simulink model "heli_p4_kalman_kf_r2020b"  (R2020b)
settings: Solver=ode1  StartTime=0.0  StopTime=45  FixedStep=0.002  RelTol=1e-3  EnableMultiTasking=on
PostLoadFcn:
  | qc_set_target_type(getConfigSet(bdroot, 'QUARC Default Target Configuration'));
values from neighbouring files (symbols this model uses):
  Ad = sys_kf.A    [p4_kalman.m]
  Bd = sys_kf.B    [p4_kalman.m]
  Cd = sys_kf.C    [p4_kalman.m]
  e_offset = heli_e_offset()    [heli_params.m]
  F = zeros(2)    [p4_controller.m]    (also in p4_kalman.m = zeros(size(F)))
  Joystick_gain_x = 1    [init_heli_3_10.m]
  Joystick_gain_y = -1    [init_heli_3_10.m]
  K = lqr(A_lqri, B_lqri, Q, R)    [p4_controller.m]    (also in p4_kalman.m = zeros(size(K)); p4_report_figs.m = floor((numel(x) - N)/step) + 1; p4_report_figs_backup_20261114.m = floor((numel(x) - N)/step) + 1; p4_report_figs_backup_before_qd_limits.m = floor((numel(x) - N)/step) + 1)
  P0 = eye(6)    [p4_kalman.m]
  Qd = Qd_vl    [p4_kalman.m]
  Rd = [0.00131511792463 0.00165099561417 0.00239206219708 -0.000707556992436 -6.43652106551e-05 0.00165099561417 0.0114715333934 0.0157536439693 -0.00145108778115 -0.000320746387433 0.00239206219708 0.0157536439693 ... (25 elements, 5x5)]    [Rd_flying.mat]    (also in p4_kalman.m = diag([1e-3 1e-3 1e-3 1e-3 1e-3]); p4_noise.m = R_hover)
  Vs0 = 7.3    [heli_params.m]    (also in p4_kalman.m = 0)
  x0 = zeros(6,1)    [p4_kalman.m]
undefined symbols (not defined in the file or in its folder): HIL, qc_get_step_size
libraries: quarc_library x9
settings Model: SimulationMode=external  ExtModeTrigDuration=60000  Creator=Rchan  LastModifiedBy=thorof
settings SolverCC: PositivePriorityOrder=on
settings DataIOCC: LimitDataPoints=on  SaveFormat=Array  SignalLoggingSaveFormat=ModelDataLogs  ReturnWorkspaceOutputs=off
settings OptimizationCC: ExpressionDepthLimit=2147483647  InitFltsAndDblsToZero=on  LifeSpan=inf
settings DebuggingCC: SaveWithParameterizedLinksMsg=none  UnderspecifiedInitializationDetection=Classic  MergeDetectMultiDrivingBlocksExec=none  SolverPrmCheckMsg=warning  MultiTaskDSMMsg=warning  MultiTaskCondExecSysMsg=none  FcnCallInpInsideContextMsg=warning  AllowSymbolicDim=off  StateNameClashWarn=warning  SFUnexpectedBacktrackingDiag=warning  SFNoUnconditionalDefaultTransitionDiag=warning  SFExecutionAtInitializationDiag=none  ArithmeticOperatorsInVariantConditions=warning
settings HardwareCC: ProdBitPerPointer=32  ProdBitPerSizeT=32  ProdBitPerPtrDiffT=32  ProdLargestAtomicFloat=None  ProdIntDivRoundTo=Undefined  ProdEndianess=Unspecified  ProdWordSize=32  ProdHWDeviceType=32-bit Generic
settings ModelReferenceCC: PropagateSignalLabelsOutOfModel=off
settings SFSimCC: SimUseLocalCustomCode=off  CustomCodeUndefinedFunction=UseInterfaceOnly
settings RTWCC: Description=QUARC Win64 Target  SystemTargetFile=quarc_win64.tlc  TemplateMakefile=quarc_default_tmf  RTWUseLocalCustomCode=off
settings CodeAppCC: StateflowObjectComments=on
settings GRTTargetCC: TargetLangStandard=C89/C90 (ANSI)  ParMdlRefBuildCompliant=off  CompOptLevelCompliant=off  CombineOutputUpdateFcns=off  MatFileLogging=off  GRTInterface=on  UseToolchainInfoCompliant=off  ExtMode=on  ExtModeMexFile=quarc_comm
settings ConfigComp: CovMetricSettings=dw  CovSaveCumulativeToWorkspaceVar=on  CovSaveSingleToWorkspaceVar=on  CovExternalEMLEnable=off  CovSFcnEnable=off

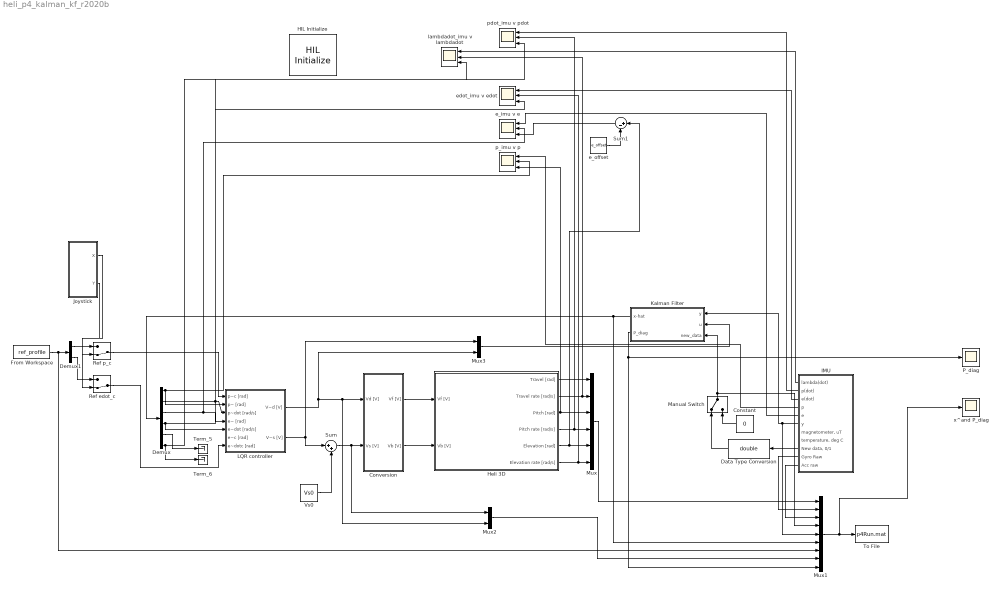
== system heli_p4_kalman_kf_r2020b ==
  Constant : Constant  Value=0
  Conversion : Subsystem
  Data Type Conversion : DataTypeConversion  OutDataTypeStr=double
  Demux : Demux  Outputs=6
  Demux1 : Demux  Outputs=2
  From Workspace : FromWorkspace  VariableName=ref_profile  SampleTime=0.002  OutputAfterFinalValue=Holding final value
  HIL Initialize : quarc_library/Data Acquisition/Generic/Configuration/HIL Initialize  Priority=-99  object_name=HIL-1  board_type=q8_usb  board_number=0  board_options=update_rate=normal;decimation=1  exclusive=off  active=off  hardware_clocks=[0:2]  clock_modes=[]  initial_clock_frequencies=[]  set_clock_params_at_start=off  set_clock_params_at_switch_in=off  set_clock_frequencies_at_start=off  set_clock_frequencies_at_switch_in=off  analog_input_channels=[0:7]  analog_input_configurations=[]  analog_input_maximums=10  analog_input_minimums=-10  set_analog_input_params_at_start=on  set_analog_input_params_at_switch_in=off  analog_output_channels=[0:7]  analog_output_maximums=10  analog_output_minimums=-10  initial_analog_outputs=[0]  final_analog_outputs=[0]  watchdog_analog_outputs=0  set_analog_output_params_at_start=on  set_analog_output_params_at_switch_in=off  set_analog_outputs_at_start=on  set_analog_outputs_at_switch_in=off  set_analog_outputs_at_terminate=on  set_analog_outputs_at_switch_out=off  set_analog_outputs_on_watchdog=off  digital_input_channels=[]  digital_output_channels=[]  digital_output_configuration=[]  initial_digital_outputs=[1]  final_digital_outputs=[1]  watchdog_digital_outputs=[1]  set_digital_output_params_at_start=off  set_digital_output_params_at_switch_in=off  set_digital_outputs_at_start=on  set_digital_outputs_at_switch_in=off  set_digital_outputs_at_terminate=on  set_digital_outputs_at_switch_out=off  set_digital_outputs_on_watchdog=off  encoder_channels=[0:7]  quadrature=[4]  encoder_filter_frequency=[]  initial_encoder_counts=[0]  set_encoder_params_at_start=on  set_encoder_params_at_switch_in=off  set_encoder_counts_at_start=on  set_encoder_counts_at_switch_in=off  pwm_channels=[0:7]  pwm_modes=0  pwm_frequency=99.532799999999995e6/4095  pwm_configuration=[0]  pwm_alignment=[0]  pwm_polarity=[1]  pwm_leading_deadband=[0]  pwm_trailing_deadband=[0]  initial_pwm_outputs=[0]  final_pwm_outputs=[0]  watchdog_pwm_outputs=[0]  set_pwm_params_at_start=on  set_pwm_params_at_switch_in=off  set_pwm_outputs_at_start=on  set_pwm_outputs_at_switch_in=off  set_pwm_outputs_at_terminate=on  set_pwm_outputs_at_switch_out=off  set_pwm_outputs_on_watchdog=off  other_output_channels=[]  initial_other_outputs=[]  final_other_outputs=[]  watchdog_other_outputs=[]  set_other_outputs_at_start=off  set_other_outputs_at_switch_in=off  set_other_outputs_at_terminate=off  set_other_outputs_at_switch_out=off  set_other_outputs_on_watchdog=off
  Heli 3D : Subsystem
  IMU : Subsystem
  Joystick : Subsystem
  Kalman Filter : Subsystem
  LQR controller : Subsystem
  Manual Switch : ManualSwitch
  Mux : Mux  Inputs=6
  Mux1 : Mux  Inputs=9
  Mux2 : Mux  Inputs=2
  Mux3 : Mux  Inputs=2
  P_diag : Scope
  Ref edot_c : ManualSwitch  CurrentSetting=0
  Ref p_c : ManualSwitch  CurrentSetting=0
  Sum : Sum  Inputs=|++
  Sum1 : Sum  Inputs=|+-
  Term_5 : Terminator
  Term_6 : Terminator
  To File : ToFile  Filename=p4Run.mat
  Vs0 : Constant  Value=Vs0
  e_imu v e : Scope  NumInputPorts=3
  e_offset : Constant  Value=e_offset
  edot_imu v edot : Scope  NumInputPorts=3
  lambdadot_imu v lambdadot : Scope  NumInputPorts=3
  p_imu v p : Scope  NumInputPorts=3
  pdot_imu v pdot : Scope  NumInputPorts=3
  x^and P_diag : Scope
  wires:
  Conversion/2(Vb [V]) -> Heli 3D/2(Vb [V])
  Conversion/1(Vf [V]) -> Heli 3D/1(Vf [V])
  Heli 3D/1(Travel [rad]) -> Mux/1
  Mux/1 -> Mux1/1
  Heli 3D/6(Elevation rate [rad/s]) -> edot_imu v edot/2, Mux/6
  Heli 3D/3(Pitch [rad]) -> p_imu v p/3, Mux/3
  Heli 3D/2(Travel rate [rad/s]) -> lambdadot_imu v lambdadot/2, Mux/2
  Heli 3D/4(Pitch rate [rad/s]) -> pdot_imu v pdot/2, Mux/4
  Heli 3D/5(Elevation [rad]) -> Sum1/1, Mux/5
  IMU/1(lambda(dot)) -> lambdadot_imu v lambdadot/1
  IMU/2(p(dot)) -> pdot_imu v pdot/1
  IMU/3(e(dot)) -> edot_imu v edot/1
  IMU/4(p) -> p_imu v p/1
  IMU/5(e) -> e_imu v e/1
  Mux1/1 -> x^and P_diag/1, To File/1
  IMU/10(Gyro Raw) -> Mux1/2
  IMU/11(Acc raw) -> Mux1/3
  IMU/6(y) -> Kalman Filter/1(y), Mux1/5
  LQR controller/1(V~d [V]) -> Mux3/2, Mux2/2, Conversion/1(Vd [V])
  LQR controller/2(V~s [V]) -> Mux3/1, Sum/1
  Demux/1 -> p_imu v p/2, LQR controller/2(p~ [rad])
  Demux/2 -> LQR controller/3(p~dot [rad/s]), pdot_imu v pdot/3
  Vs0/1 -> Sum/2
  Sum/1 -> Mux2/1, Conversion/2(Vs [V])
  From Workspace/1 -> Mux1/7, Demux1/1
  Mux2/1 -> Mux1/8
  Demux/4 -> LQR controller/5(e~dot [rad/s]), edot_imu v edot/3
  IMU/9("New data, 0/1") -> Data Type Conversion/1
  Data Type Conversion/1 -> Manual Switch/1
  Constant/1 -> Manual Switch/2
  Manual Switch/1 -> Kalman Filter/3(new_data), Mux1/4
  Mux3/1 -> Kalman Filter/2(u)
  Kalman Filter/1(x-hat) -> Demux/1, Mux1/6
  Demux/3 -> e_imu v e/2, LQR controller/4(e~ [rad])
  Demux/5 -> Term_5/1
  Demux/6 -> Term_6/1, lambdadot_imu v lambdadot/3
  Kalman Filter/2(P_diag) -> Mux1/9, P_diag/1
  Demux1/1 -> Ref p_c/1
  Joystick/1(X) -> Ref p_c/2
  Ref p_c/1 -> LQR controller/1(p~c [rad])
  Demux1/2 -> Ref edot_c/1
  Joystick/2(Y) -> Ref edot_c/2
  Ref edot_c/1 -> LQR controller/7(e~dotc [rad])
  e_offset/1 -> Sum1/2
  Sum1/1 -> e_imu v e/3

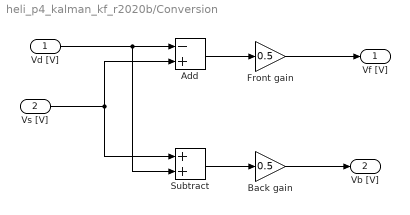
== system heli_p4_kalman_kf_r2020b/Conversion ==
  Vd [V] : Inport
  Vs [V] : Inport  Port=2
  Add : Sum  Inputs=-+
  Back gain : Gain  Gain=0.5
  Front gain : Gain  Gain=0.5
  Subtract : Sum
  Vf [V] : Outport
  Vb [V] : Outport  Port=2
  wires:
  Vd [V]/1 -> Subtract/2, Add/1
  Vs [V]/1 -> Subtract/1, Add/2
  Subtract/1 -> Back gain/1
  Back gain/1 -> Vb [V]/1
  Add/1 -> Front gain/1
  Front gain/1 -> Vf [V]/1

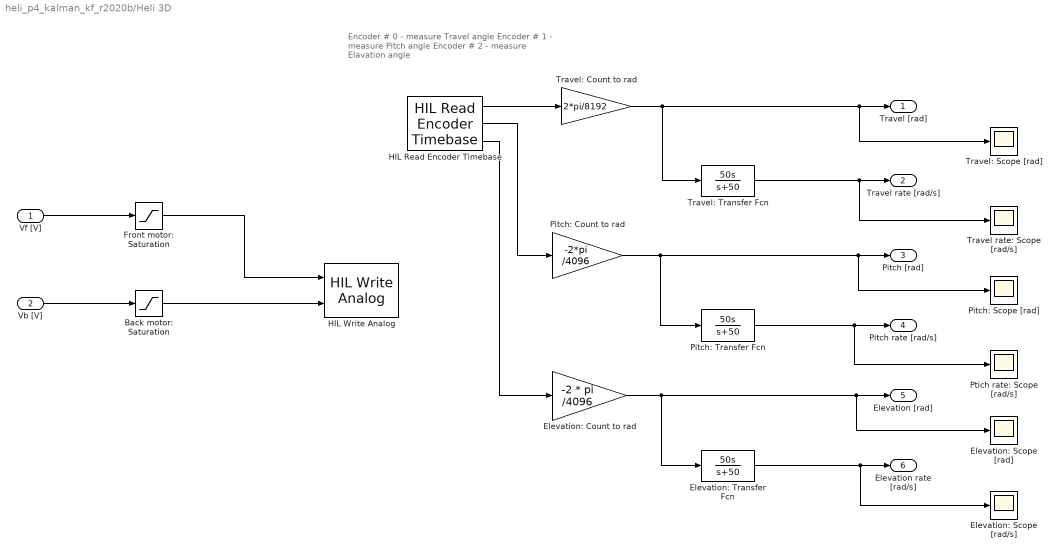
== system heli_p4_kalman_kf_r2020b/Heli 3D ==
  note: Encoder # 0 - measure Travel angle
      | Encoder # 1 - measure Pitch angle
      | Encoder # 2 - measure Elavation angle
  Vf [V] : Inport
  Vb [V] : Inport  Port=2
  Back motor: Saturation : Saturate  UpperLimit=5  LowerLimit=-5
  Elevation: Count to rad : Gain  Gain=-2 * pi /4096
  Elevation: Scope [rad/s] : Scope
  Elevation: Scope [rad] : Scope
  Elevation: Transfer Fcn : TransferFcn  Numerator=[50 0]  Denominator=[1 50]
  Front motor: Saturation : Saturate  UpperLimit=5  LowerLimit=-5
  HIL Read Encoder Timebase : quarc_library/Data Acquisition/Generic/Timebases/HIL Read Encoder Timebase  object_name=HIL-1  clock=0  channels=[0:2]  active=on  vector_output=off  data_type_mode=Inherit via back propagation  data_type=double  overflow_mode=Error on overflow  samples_in_buffer=max(ceil(1/qc_get_step_size), 1)
  HIL Write Analog : quarc_library/Data Acquisition/Generic/Immediate I//O/HIL Write Analog  object_name=HIL-1  channels=[0:1]  sample_time=-1  active=off  vector_input=off
  Pitch: Count to rad : Gain  Gain=-2*pi /4096
  Pitch: Scope [rad] : Scope
  Pitch: Transfer Fcn : TransferFcn  Numerator=[50 0]  Denominator=[1 50]
  Ptich rate: Scope [rad/s] : Scope
  Travel rate: Scope [rad/s] : Scope
  Travel: Count to rad : Gain  Gain=2*pi/8192
  Travel: Scope [rad] : Scope
  Travel: Transfer Fcn : TransferFcn  Numerator=[50 0]  Denominator=[1 50]
  Travel [rad] : Outport
  Travel rate [rad/s] : Outport  Port=2
  Pitch [rad] : Outport  Port=3
  Pitch rate [rad/s] : Outport  Port=4
  Elevation [rad] : Outport  Port=5
  Elevation rate [rad/s] : Outport  Port=6
  wires:
  HIL Read Encoder Timebase/1 -> Travel: Count to rad/1
  HIL Read Encoder Timebase/2 -> Pitch: Count to rad/1
  HIL Read Encoder Timebase/3 -> Elevation: Count to rad/1
  Travel: Count to rad/1 -> Travel: Scope [rad]/1, Travel [rad]/1, Travel: Transfer Fcn/1
  Travel: Transfer Fcn/1 -> Travel rate: Scope [rad/s]/1, Travel rate [rad/s]/1
  Pitch: Count to rad/1 -> Pitch: Transfer Fcn/1, Pitch: Scope [rad]/1, Pitch [rad]/1
  Pitch: Transfer Fcn/1 -> Ptich rate: Scope [rad/s]/1, Pitch rate [rad/s]/1
  Elevation: Count to rad/1 -> Elevation: Transfer Fcn/1, Elevation: Scope [rad]/1, Elevation [rad]/1
  Elevation: Transfer Fcn/1 -> Elevation: Scope [rad/s]/1, Elevation rate [rad/s]/1
  Vf [V]/1 -> Front motor: Saturation/1
  Vb [V]/1 -> Back motor: Saturation/1
  Front motor: Saturation/1 -> HIL Write Analog/1
  Back motor: Saturation/1 -> HIL Write Analog/2

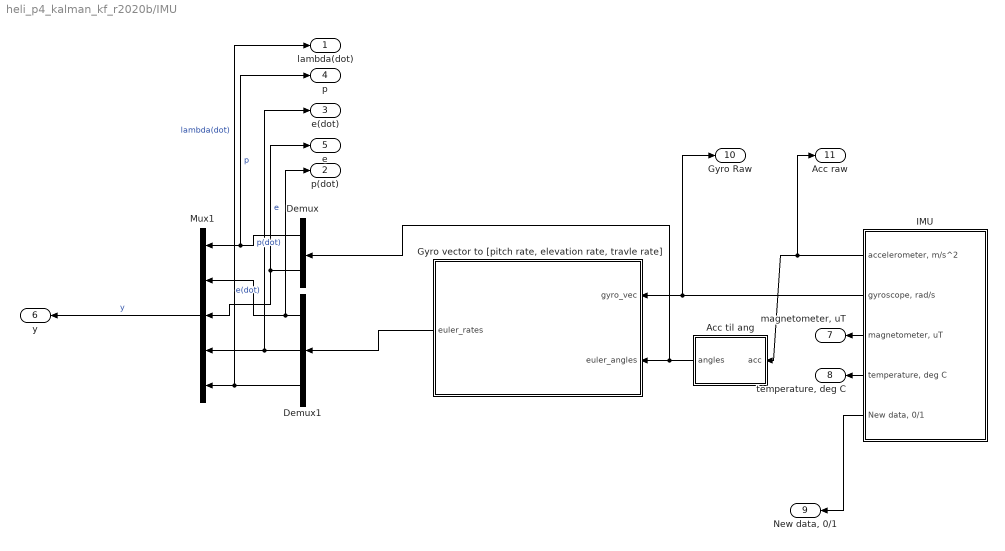
== system heli_p4_kalman_kf_r2020b/IMU ==
  Acc til ang : MATLAB Function  TreatAsAtomicUnit=on
  Demux : Demux  Outputs=2
  Demux1 : Demux  Outputs=3
  "Gyro vector to [pitch rate, elevation rate, travle rate]" : MATLAB Function  TreatAsAtomicUnit=on
  IMU : Subsystem
  Mux1 : Mux  Inputs=5
  lambda(dot) : Outport
  p(dot) : Outport  Port=2
  e(dot) : Outport  Port=3
  p : Outport  Port=4
  e : Outport  Port=5
  y : Outport  Port=6
  "magnetometer, uT" : Outport  Port=7
  "temperature, deg C" : Outport  Port=8
  "New data, 0/1" : Outport  Port=9
  Gyro Raw : Outport  Port=10
  Acc raw : Outport  Port=11
  wires:
  IMU/1("accelerometer, m/s^2") -> Acc raw/1, Acc til ang/1(acc)
  Demux1/3 -> lambda(dot)/1, Mux1/5  "lambda(dot)"
  "Gyro vector to [pitch rate, elevation rate, travle rate]"/1(euler_rates) -> Demux1/1
  IMU/2("gyroscope, rad/s") -> Gyro Raw/1, "Gyro vector to [pitch rate, elevation rate, travle rate]"/1(gyro_vec)
  Demux/1 -> p/1, Mux1/1  "p"
  Demux1/1 -> p(dot)/1, Mux1/2  "p(dot)"
  Demux1/2 -> e(dot)/1, Mux1/4  "e(dot)"
  Mux1/1 -> y/1  "y"
  Demux/2 -> e/1, Mux1/3  "e"
  IMU/5("New data, 0/1") -> "New data, 0/1"/1
  IMU/3("magnetometer, uT") -> "magnetometer, uT"/1
  IMU/4("temperature, deg C") -> "temperature, deg C"/1
  Acc til ang/1(angles) -> Demux/1, "Gyro vector to [pitch rate, elevation rate, travle rate]"/2(euler_angles)

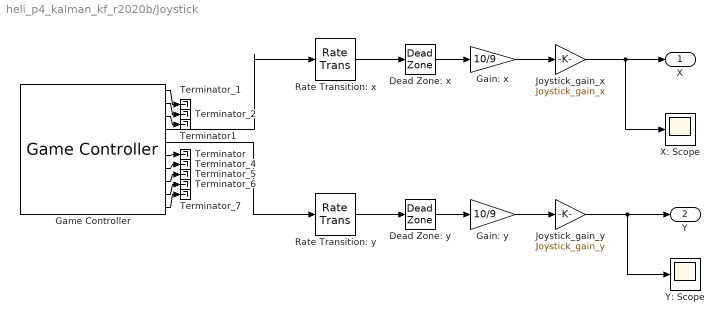
== system heli_p4_kalman_kf_r2020b/Joystick ==
  Dead Zone: x : DeadZone  LowerValue=-0.1  UpperValue=0.1  SaturateOnIntegerOverflow=on
  Dead Zone: y : DeadZone  LowerValue=-0.1  UpperValue=0.1  SaturateOnIntegerOverflow=on
  Gain: x : Gain  Gain=10/9
  Gain: y : Gain  Gain=10/9
  Game Controller : quarc_library/Devices/Peripherals/Target/Game Controller  controller=1  buffer_size=12  deadzone=[]  saturation=[]  sample_time=max(qc_get_step_size, 0.01)  auto_center=off  enabled=on
      settings: SourceProductName=QUARC Targets
  Joystick_gain_x : Gain  Gain=Joystick_gain_x
  Joystick_gain_y : Gain  Gain=Joystick_gain_y
  Rate Transition: x : RateTransition
  Rate Transition: y : RateTransition
  Terminator : Terminator
  Terminator1 : Terminator
  Terminator_{1..2,4..7} (6 alike) : Terminator
  X: Scope : Scope
  Y: Scope : Scope
  X : Outport
  Y : Outport  Port=2
  wires:
  Rate Transition: y/1 -> Dead Zone: y/1
  Rate Transition: x/1 -> Dead Zone: x/1
  Game Controller/5 -> Rate Transition: y/1
  Game Controller/4 -> Rate Transition: x/1
  Game Controller/1 -> Terminator_1/1
  Game Controller/2 -> Terminator_2/1
  Game Controller/7 -> Terminator_4/1
  Game Controller/8 -> Terminator_5/1
  Game Controller/9 -> Terminator_6/1
  Game Controller/10 -> Terminator_7/1
  Game Controller/3 -> Terminator1/1
  Game Controller/6 -> Terminator/1
  Dead Zone: x/1 -> Gain: x/1
  Dead Zone: y/1 -> Gain: y/1
  Gain: x/1 -> Joystick_gain_x/1
  Gain: y/1 -> Joystick_gain_y/1
  Joystick_gain_x/1 -> X/1, X: Scope/1
  Joystick_gain_y/1 -> Y: Scope/1, Y/1

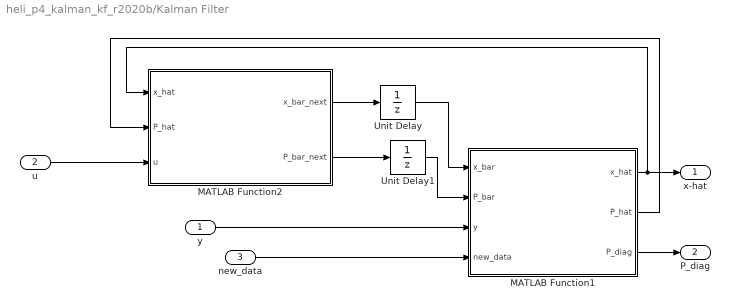
== system heli_p4_kalman_kf_r2020b/Kalman Filter ==
  y : Inport
  u : Inport  Port=2
  new_data : Inport  Port=3
  MATLAB Function1 : MATLAB Function  TreatAsAtomicUnit=on
  MATLAB Function2 : MATLAB Function  TreatAsAtomicUnit=on
  Unit Delay : UnitDelay  InitialCondition=x0  SampleTime=0.002  HasFrameUpgradeWarning=on
  Unit Delay1 : UnitDelay  InitialCondition=P0  SampleTime=-1  HasFrameUpgradeWarning=on
  x-hat : Outport
  P_diag : Outport  Port=2
  wires:
  MATLAB Function2/1(x_bar_next) -> Unit Delay/1
  MATLAB Function2/2(P_bar_next) -> Unit Delay1/1
  y/1 -> MATLAB Function1/3(y)
  Unit Delay/1 -> MATLAB Function1/1(x_bar)
  Unit Delay1/1 -> MATLAB Function1/2(P_bar)
  u/1 -> MATLAB Function2/3(u)
  MATLAB Function1/1(x_hat) -> MATLAB Function2/1(x_hat), x-hat/1
  new_data/1 -> MATLAB Function1/4(new_data)
  MATLAB Function1/2(P_hat) -> MATLAB Function2/2(P_hat)
  MATLAB Function1/3(P_diag) -> P_diag/1

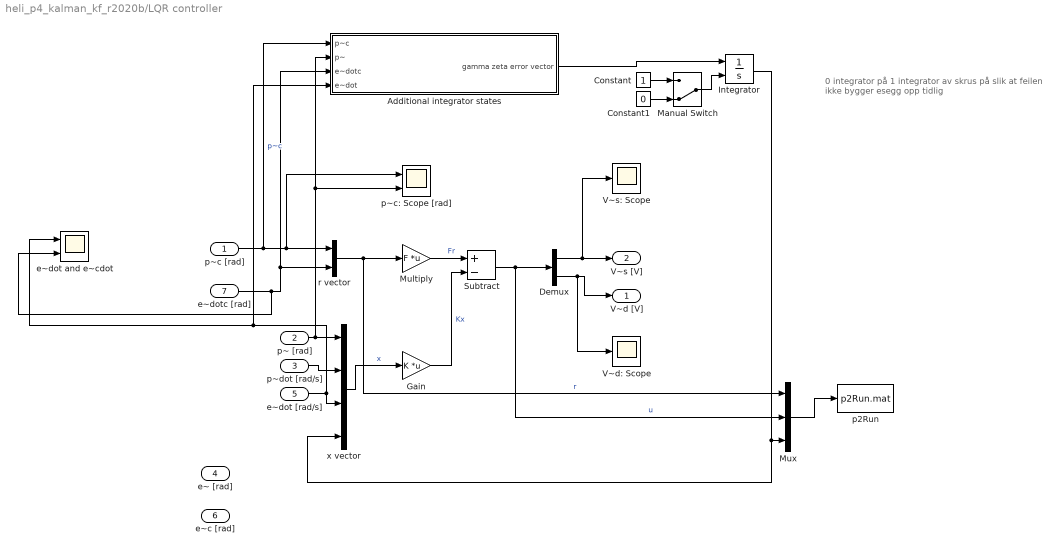
== system heli_p4_kalman_kf_r2020b/LQR controller ==
  note: 0 integrator på
      | 1 integrator av
      | skrus på slik at feilen ikke bygger esegg opp tidlig
  p~c [rad] : Inport
  p~ [rad] : Inport  Port=2
  p~dot [rad/s] : Inport  Port=3
  e~ [rad] : Inport  Port=4
  e~dot [rad/s] : Inport  Port=5
  e~c [rad] : Inport  Port=6
  e~dotc [rad] : Inport  Port=7
  Additional integrator states : Subsystem
  Constant : Constant
  Constant1 : Constant  Value=0
  Demux : Demux  Outputs=2
  Gain : Gain  Gain=K  Multiplication=Matrix(K*u)
  Integrator : Integrator  ExternalReset=level
  Manual Switch : ManualSwitch  CurrentSetting=0
  Multiply : Gain  Gain=F  Multiplication=Matrix(K*u)
  Mux : Mux  Inputs=3
  Subtract : Sum  Inputs=+-
  V~d: Scope : Scope
  V~s: Scope : Scope
  e~dot and e~cdot : Scope  NumInputPorts=2
  p2Run : ToFile  Filename=p2Run.mat
  p~c: Scope [rad] : Scope  NumInputPorts=2
  r vector : Mux  Inputs=2
  x vector : Mux
  V~d [V] : Outport  InitialOutput=0
  V~s [V] : Outport  Port=2  InitialOutput=0
  wires:
  p~c [rad]/1 -> Additional integrator states/1(p~c), p~c: Scope [rad]/1, r vector/1  "p~c"
  e~dotc [rad]/1 -> e~dot and e~cdot/2, r vector/2, Additional integrator states/3(e~dotc)
  r vector/1 -> Mux/1, Multiply/1  "r"
  Multiply/1 -> Subtract/1  "Fr"
  x vector/1 -> Gain/1  "x"
  Gain/1 -> Subtract/2  "Kx"
  e~dot [rad/s]/1 -> Additional integrator states/4(e~dot), e~dot and e~cdot/1, x vector/3
  p~ [rad]/1 -> Additional integrator states/2(p~), p~c: Scope [rad]/2, x vector/1
  p~dot [rad/s]/1 -> x vector/2
  Subtract/1 -> Mux/2, Demux/1  "u"
  Demux/1 -> V~s: Scope/1, V~s [V]/1
  Demux/2 -> V~d: Scope/1, V~d [V]/1
  Mux/1 -> p2Run/1
  Additional integrator states/1(gamma zeta error vector) -> Integrator/1
  Integrator/1 -> Mux/3, x vector/4
  Manual Switch/1 -> Integrator/2
  Constant/1 -> Manual Switch/1
  Constant1/1 -> Manual Switch/2

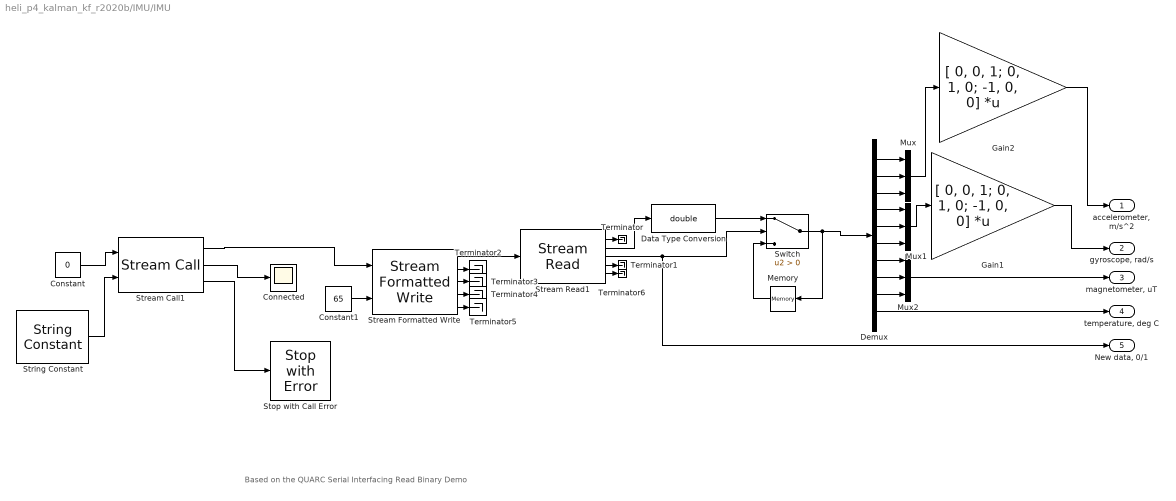
== system heli_p4_kalman_kf_r2020b/IMU/IMU ==
  note: Based on the QUARC Serial Interfacing Read Binary Demo
  Connected : Scope
  Constant : Constant  Value=0
  Constant1 : Constant  Value=65
  Data Type Conversion : DataTypeConversion  OutDataTypeStr=double
  Demux : Demux  Outputs=10
  Gain1 : Gain  Gain=[ 0, 0, 1; 0, 1, 0; -1, 0, 0]  Multiplication=Matrix(K*u) (u vector)
  Gain2 : Gain  Gain=[ 0, 0, 1; 0, 1, 0; -1, 0, 0]  Multiplication=Matrix(K*u) (u vector)
  Memory : Memory  InitialCondition=[0 0 0 0 0 0 0 0 0 0]
  Mux : Mux  Inputs=3
  Mux1 : Mux  Inputs=3
  Mux2 : Mux  Inputs=3
  Stop with Call Error : quarc_library/Sinks/Error Handling/Stop with Error  message_type=Interpret input as error code  message=Error occurred
      settings: SourceProductName=QUARC Targets
  Stream Call1 : quarc_library/Communications/Intermediate/Stream Call  uri_source=External input port  uri=serial://IMU:9?baud=115200,word=8,parity=none,stop=1,flow='none'  apply_uri_to_all_configs=on  send_buffer_size=8000  receive_buffer_size=8000  byte_order=little endian (Intel - LSB first)  sample_time=qc_get_step_size  non_blocking=on  active=off
      settings: SourceProductName=QUARC Targets
  Stream Formatted Write : quarc_library/Communications/Intermediate/Stream Formatted Write  format_string=%c\n  max_code_units=80  optimization=Minimizing latency
      settings: SourceProductName=QUARC Targets
  Stream Read1 : quarc_library/Communications/Intermediate/Stream Read  data_type=single  type_expr=BusObject  num_elements=10  receive_dims=off
      settings: SourceProductName=QUARC Targets
  String Constant : quarc_library/Strings/String Constant  string_value=qc_perform_substitutions('serial://IMU:%{PORT}?baud=115200,word=8,parity=none,stop=1')  evaluate_string=on  string_type=URI  max_length=255  sample_time=inf  variable_size=off
      settings: AttributesFormatString="\"serial://IMU:4?baud=115200,word=8,parity=none,stop=1\""  SourceProductName=QUARC Targets
  Switch : Switch  Criteria=u2 > Threshold
  Terminator{,1..6} (7 alike) : Terminator
  "accelerometer, m/s^2" : Outport
  "gyroscope, rad/s" : Outport  Port=2
  "magnetometer, uT" : Outport  Port=3
  "temperature, deg C" : Outport  Port=4
  "New data, 0/1" : Outport  Port=5
  wires:
  Switch/1 -> Memory/1, Demux/1
  Data Type Conversion/1 -> Switch/1
  Stream Read1/3 -> "New data, 0/1"/1, Switch/2
  Stream Formatted Write/1 -> Stream Read1/1
  Constant1/1 -> Stream Formatted Write/2
  Gain1/1 -> "gyroscope, rad/s"/1
  Gain2/1 -> "accelerometer, m/s^2"/1
  Stream Read1/4 -> Terminator1/1
  Demux/10 -> "temperature, deg C"/1
  Mux1/1 -> Gain1/1
  Stream Read1/2 -> Data Type Conversion/1
  Demux/7 -> Mux2/1
  Demux/8 -> Mux2/2
  Demux/9 -> Mux2/3
  Mux2/1 -> "magnetometer, uT"/1
  Demux/6 -> Mux1/3
  Demux/5 -> Mux1/2
  Demux/4 -> Mux1/1
  Mux/1 -> Gain2/1
  Demux/3 -> Mux/3
  Demux/1 -> Mux/1
  Demux/2 -> Mux/2
  Stream Read1/1 -> Terminator/1
  Stream Call1/1 -> Stream Formatted Write/1
  Constant/1 -> Stream Call1/1
  String Constant/1 -> Stream Call1/2
  Stream Call1/2 -> Connected/1
  Stream Call1/3 -> Stop with Call Error/1
  Memory/1 -> Switch/3
  Stream Formatted Write/2 -> Terminator2/1
  Stream Formatted Write/3 -> Terminator3/1
  Stream Formatted Write/4 -> Terminator4/1
  Stream Formatted Write/5 -> Terminator5/1
  Stream Read1/5 -> Terminator6/1

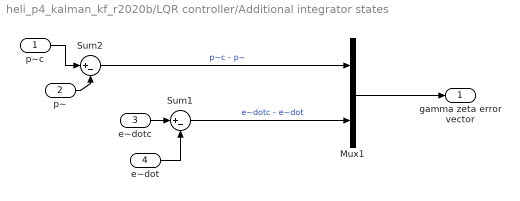
== system heli_p4_kalman_kf_r2020b/LQR controller/Additional integrator states ==
  p~c : Inport
  p~ : Inport  Port=2
  e~dotc : Inport  Port=3
  e~dot : Inport  Port=4
  Mux1 : Mux  Inputs=2
  Sum1 : Sum  Inputs=|+-
  Sum2 : Sum  Inputs=|+-
  gamma zeta error vector : Outport
  wires:
  p~c/1 -> Sum2/1
  Sum2/1 -> Mux1/1  "p~c - p~"
  p~/1 -> Sum2/2
  Mux1/1 -> gamma zeta error vector/1
  Sum1/1 -> Mux1/2  "e~dotc - e~dot"
  e~dotc/1 -> Sum1/1
  e~dot/1 -> Sum1/2

== matlab function heli_p4_kalman_kf_r2020b/IMU/Acc til ang ==
  data: acc input; angles output
function angles = acc_to_angles(acc)
    ax = acc(1); ay = acc(2); az = acc(3);
    p = atan2(-ay, -az);
    e = atan2(ax, sqrt(ay^2 + az^2));
    angles = [p; e];
end

== matlab function heli_p4_kalman_kf_r2020b/IMU/Gyro vector to [pitch rate, elevation rate, travle rate] ==
  data: gyro_vec input; euler_rates output; euler_angles input
function euler_rates = gyro_vec_to_euler_rates(gyro_vec,euler_angles)
%#codegen
    phi = euler_angles(1);    % p
    theta = euler_angles(2);  % e

     %phi = max(min(euler_angles(1), deg2rad(80)), -deg2rad(80));    % p
     %theta = max(min(euler_angles(2), deg2rad(80)), -deg2rad(80));  % e


    T = [1, sin(phi)*tan(theta), cos(phi)*tan(theta);
         0, cos(phi),            -sin(phi);
         0, sin(phi)/cos(theta), cos(phi)/cos(theta)]; 
    
euler_rates = T*gyro_vec;

== matlab function heli_p4_kalman_kf_r2020b/Kalman Filter/MATLAB Function1 ==
  data: x_bar input; x_hat output; P_bar input; y input; new_data input; P_hat output; P_diag output; Cd parameter; Rd parameter
function [x_hat, P_hat, P_diag] = kf_correct(x_bar, P_bar, y, new_data, Cd, Rd)
% KF_CORRECT  Correction step (2.21a-c), only when new IMU data has arrived.
%   Paste into a MATLAB Function block.
%   Inputs  (signals)   : x_bar [n x 1], P_bar [n x n] (from the Unit Delays),
%                         y [5 x 1] IMU measurement, new_data (0/1, via Manual Switch)
%   Inputs  (Parameter) : Cd, Rd
%   Outputs             : x_hat, P_hat (to controller + kf_predict),
%                         P_diag = diag(P_hat) for scopes / logging
%
%   No new data:  x_hat = x_bar,  P_hat = P_bar   (eq. 2.2-2.3 in the assignment)
%#codegen
n = numel(x_bar);
if new_data > 0.5
    S     = Cd*P_bar*Cd.' + Rd;
    L     = (P_bar*Cd.') / S;                       % Kalman gain
    x_hat = x_bar + L*(y - Cd*x_bar);
    IKC   = eye(n) - L*Cd;
    P_hat = IKC*P_bar*IKC.' + L*Rd*L.';             % Joseph form
    P_hat = 0.5*(P_hat + P_hat.');
else
    x_hat = x_bar;
    P_hat = P_bar;
end
P_diag = diag(P_hat);
end

== matlab function heli_p4_kalman_kf_r2020b/Kalman Filter/MATLAB Function2 ==
  data: x_hat input; P_hat input; u input; x_bar_next output; P_bar_next output; Ad parameter; Bd parameter; Qd parameter
function [x_bar_next, P_bar_next] = kf_predict(x_hat, P_hat, u, Ad, Bd, Qd)
% KF_PREDICT  Prediction step (2.21d-e). Paste into a MATLAB Function block.
%   Inputs  (signals)   : x_hat [n x 1], P_hat [n x n], u = [Vs_tilde; Vd]
%   Inputs  (Parameter) : Ad, Bd, Qd   (set Scope = Parameter in the Symbols
%                         pane / Ports & Data Manager so they are read from
%                         the workspace created by p4_kalman.m)
%   Outputs             : x_bar[k+1], P_bar[k+1]  -> Unit Delay -> kf_correct
%#codegen
x_bar_next = Ad*x_hat + Bd*u;
P_bar_next = Ad*P_hat*Ad.' + Qd;
P_bar_next = 0.5*(P_bar_next + P_bar_next.');     % keep symmetric numerically
end
